simulink model "ECM_1RC_simulink_LUT"  (R2025b)
settings: Solver=ode23t  StartTime=0.0  StopTime=3600  MaxStep=1  RelTol=1e-3
values from neighbouring files (symbols this model uses):
  C1_sim = [35.3076805194 14.2971811644 613.99886549 1179.36911146 1456.66608606 1589.99406408 1623.51334368 1657.82009606 1295.55255927 1167.66350194 1050.27016185 866.783843467 ... (14 elements, 1x14)]    [ECM_Parameters.mat]    (also in preparer_LUT_simulink_ECM.m = interp1(SOC_f, C1_f, SOC_sim_lut, 'linear', 'extrap'))
  OCV_sim = [2.91488074462 3.28442184481 3.41414339486 3.47766982679 3.50738926719 3.53599386865 3.5985062749 3.67111036716 3.82204698001 3.89720965748 3.97533326687 4.08384541151 ... (14 elements, 1x14)]    [ECM_Parameters.mat]    (also in preparer_LUT_simulink_ECM.m = interp1(SOC_ds_s, OCV_s, SOC_sim_lut, 'pchip', 'extrap'))
  R0_sim = [0.0332041236965 0.028168314239 0.0334794052607 0.0307077032991 0.0290955136939 0.0290570705727 0.0273599181034 0.0269173406115 0.0275195159637 0.0273690512631 0.0275653828644 0.0288893126183 ... (14 elements, 1x14)]    [ECM_Parameters.mat]    (also in preparer_LUT_simulink_ECM.m = interp1(SOC_f, R0_f, SOC_sim_lut, 'linear', 'extrap'))
  R1_sim = [0.110448594775 0.0590208655475 0.0506099065009 0.0457874694283 0.0423973812151 0.0374647624298 0.0342658709557 0.0361325328683 0.0540686493611 0.0453905030939 0.0421488523784 0.0374912211225 ... (14 elements, 1x14)]    [ECM_Parameters.mat]    (also in preparer_LUT_simulink_ECM.m = interp1(SOC_f, R1_f, SOC_sim_lut, 'linear', 'extrap'))
  SOC_sim_lut = [0.05 0.1 0.15 0.2 0.25 0.3 0.4 0.5 0.6 0.699996551724 0.8 0.899996551724 ... (14 elements, 1x14)]    [ECM_Parameters.mat]    (also in preparer_LUT_simulink_ECM.m = sort(SOC_f(:))')
settings Model: Creator=SAT  LastModifiedBy=SAT

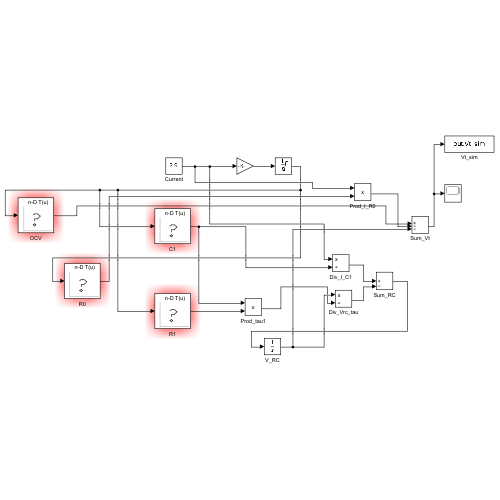
[thumbnail: Simulink's stored preview of the top-level diagram]
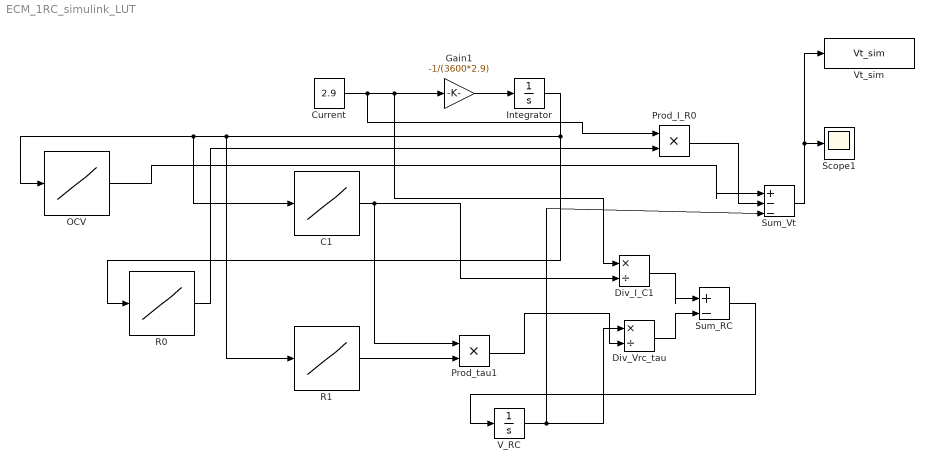
== system ECM_1RC_simulink_LUT ==
  C1 : Lookup_n-D  NumberOfTableDimensions=1  BreakpointsForDimension1=SOC_sim_lut  Table=C1_sim  InternalRulePriority=Speed  RndMeth=Simplest
  Current : Constant  Value=2.9
  Div_I_C1 : Product  Inputs=*/
  Div_Vrc_tau : Product  Inputs=*/
  Gain1 : Gain  Gain=-1/(3600*2.9)
  Integrator : Integrator  InitialCondition=1  LimitOutput=on  UpperSaturationLimit=1  LowerSaturationLimit=0
  OCV : Lookup_n-D  Description=""  NumberOfTableDimensions=1  BreakpointsForDimension1=SOC_sim_lut  Table=OCV_sim  InternalRulePriority=Speed  RndMeth=Simplest
  Prod_I_R0 : Product
  Prod_tau1 : Product
  R0 : Lookup_n-D  NumberOfTableDimensions=1  BreakpointsForDimension1=SOC_sim_lut  Table=R0_sim  InternalRulePriority=Speed  RndMeth=Simplest
  R1 : Lookup_n-D  NumberOfTableDimensions=1  BreakpointsForDimension1=SOC_sim_lut  Table=R1_sim  InternalRulePriority=Speed  RndMeth=Simplest
  Scope1 : Scope
      settings: ActiveDisplayYMinimum=1.3966572112470093  ActiveDisplayYMaximum=4.5926041927318382
  Sum_RC : Sum  Inputs=|+-
  Sum_Vt : Sum  Inputs=|+--
  V_RC : Integrator  InitialCondition=0.1140
  Vt_sim : ToWorkspace  VariableName=Vt_sim  SampleTime=-1
  wires:
  Gain1/1 -> Integrator/1
  Current/1 -> Prod_I_R0/1, Div_I_C1/1, Gain1/1
  Integrator/1 -> R1/1, C1/1, OCV/1, R0/1
  C1/1 -> Prod_tau1/1, Div_I_C1/2
  R1/1 -> Prod_tau1/2
  V_RC/1 -> Sum_Vt/3, Div_Vrc_tau/1
  Prod_tau1/1 -> Div_Vrc_tau/2
  Div_I_C1/1 -> Sum_RC/1
  Div_Vrc_tau/1 -> Sum_RC/2
  Sum_RC/1 -> V_RC/1
  R0/1 -> Prod_I_R0/2
  OCV/1 -> Sum_Vt/1
  Prod_I_R0/1 -> Sum_Vt/2
  Sum_Vt/1 -> Vt_sim/1, Scope1/1
